simulink model "thermal_control_hardware"  (R2026a)
settings: Solver=FixedStepDiscrete  StopTime=inf  FixedStep=0.1  EnableMultiTasking=on
libraries: slpidlib x1
settings Model: SimulationMode=external  SILPILModeSetting=veronly  ExtModeTrigDuration=2  Creator=Fufal Jigar  LastModifiedBy=Fufal Jigar
settings HardwareCC: ProdBitPerInt=16.0  ProdBitPerPointer=16.0  ProdBitPerSizeT=16.0  ProdBitPerPtrDiffT=16.0  ProdWordSize=8.0  ProdHWDeviceType=Atmel->AVR  UseEmbeddedCoderFeatures=off  UseSimulinkCoderFeatures=off
settings RTWCC: SystemTargetFile=ert.tlc  HardwareBoard=Arduino Mega 2560  TLCOptions=-aInlineSetEventsForThisBaseRateFcn=TLC_FALSE -aSuppressMultiTaskScheduler=TLC_FALSE -aRateBasedStepFcn=1  Toolchain=Arduino AVR  BuildConfiguration=Faster Runs  Description=Embedded Coder
settings ERTTargetCC: ExtModeTransport=3.0  ExtModeAutomaticAllocSize=off  ExtModeStaticAllocSize=2048.0  SupportContinuousTime=on  SupportNonInlinedSFcns=on  SupportVariableSizeSignals=on

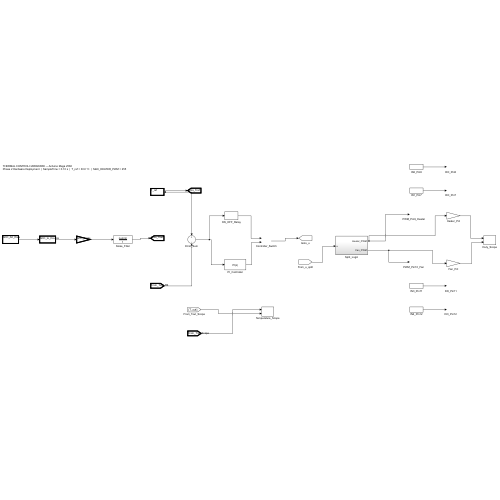
[thumbnail: Simulink's stored preview of the top-level diagram]
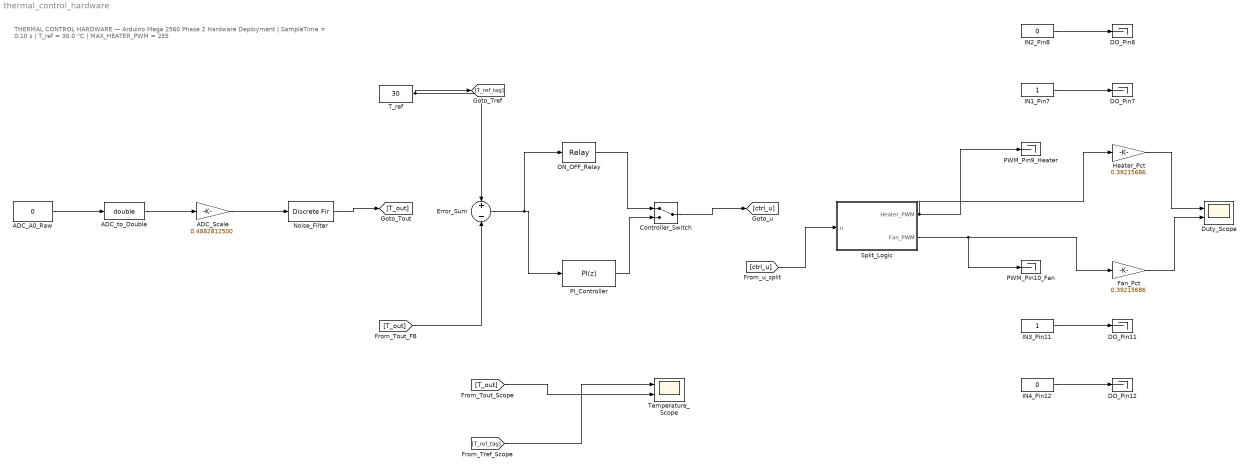
== system thermal_control_hardware ==
  note: THERMAL CONTROL HARDWARE — Arduino Mega 2560
      | Phase 2 Hardware Deployment  |  SampleTime = 0.10 s  |  T_ref = 30.0 °C  |  MAX_HEATER_PWM = 255
  ADC_A0_Raw : Constant  Value=0
  ADC_Scale : Gain  Gain=0.4882812500
  ADC_to_Double : DataTypeConversion  OutDataTypeStr=double  SaturateOnIntegerOverflow=off  RndMeth=Floor
  Controller_Switch : ManualSwitch
  DO_Pin{7..8,11..12} (4 alike) : Terminator
  Duty_Scope : Scope  NumInputPorts=2
  Error_Sum : Sum  Inputs=+-
  Fan_Pct : Gain  Gain=0.39215686
  Heater_Pct : Gain  Gain=0.39215686
  IN1_Pin7 : Constant  OutDataTypeStr=boolean
  IN2_Pin8 : Constant  Value=0  OutDataTypeStr=boolean
  IN3_Pin11 : Constant  OutDataTypeStr=boolean
  IN4_Pin12 : Constant  Value=0  OutDataTypeStr=boolean
  Noise_Filter : DiscreteFir  Coefficients=[0.2 0.2 0.2 0.2 0.2]  SampleTime=0.1
  ON_OFF_Relay : Relay  OnSwitchValue=0.5  OffSwitchValue=-0.5  OnOutputValue=255  OffOutputValue=-255
  PI_Controller : slpidlib/PID Controller  Controller=PI  Form=Parallel  TimeDomain=Discrete-time  UseExternalTs=off  SampleTime=0.1  IntegratorMethod=Forward Euler  FilterMethod=Forward Euler  ControllerParametersSource=internal  P=0.444400  I=0.003700  UseKiTs=off  D=0  UseExternalDerivativeSource=off  N=100  UseFilter=on  TunerSelectOption=Transfer Function Based (PID Tuner App)  InitialConditionSource=internal  InitialConditionForIntegrator=0  InitialConditionForFilter=0  DifferentiatorICPrevScaledInput=0  ExternalReset=none  TrackingMode=off  Kt=1  LimitOutput=off  SatLimitsSource=internal  UpperSaturationLimit=255  LowerSaturationLimit=-255  LinearizeAsGain=off  AntiWindupMode=clamping  Kb=1  LimitIntegrator=off  UpperIntegratorSaturationLimit=inf  LowerIntegratorSaturationLimit=-inf  POutMin=[]  POutMax=[]  IOutMin=[]  IOutMax=[]  DOutMin=[]  DOutMax=[]  NOutMin=[]  NOutMax=[]  SumOutMin=[]  SumOutMax=[]  SaturationOutMin=[]  SaturationOutMax=[]  PParamMin=[]  PParamMax=[]  IParamMin=[]  IParamMax=[]  DParamMin=[]  DParamMax=[]  NParamMin=[]  NParamMax=[]  KbParamMin=[]  KbParamMax=[]  KtParamMin=[]  KtParamMax=[]  KbOutMin=[]  KbOutMax=[]  KtOutMin=[]  KtOutMax=[]  IntegratorOutMin=[]  IntegratorOutMax=[]  FilterOutMin=[]  FilterOutMax=[]  SumI1OutMin=[]  SumI1OutMax=[]  SumI2OutMin=[]  SumI2OutMax=[]  SumI3OutMin=[]  SumI3OutMax=[]  SumI4OutMin=[]  SumI4OutMax=[]  SumDOutMin=[]  SumDOutMax=[]  DifferentiatorOutMin=[]  DifferentiatorOutMax=[]  FilterDiffOutCoefMin=[]  FilterDiffOutCoefMax=[]  ReciprocalOutMin=[]  ReciprocalOutMax=[]  SumDenOutMin=[]  SumDenOutMax=[]  SumNumOutMin=[]  SumNumOutMax=[]  DivideOutMin=[]  DivideOutMax=[]  UdiffTsProdOutMin=[]  UdiffTsProdOutMax=[]  NTsProdOutMin=[]  NTsProdOutMax=[]  UintegralTsProdOutMin=[]  UintegralTsProdOutMax=[]  UngainTsProdOutMin=[]  UngainTsProdOutMax=[]  ClampingZeroOutDataTypeStr=Inherit: Inherit via back propagation  ClampingZeroOutMin=[]  ClampingZeroOutMax=[]  FilterDenConstantOutDataTypeStr=Inherit: Inherit via back propagation  FilterDenConstantOutMin=[]  FilterDenConstantOutMax=[]  PCopyOutDataTypeStr=Inherit: Inherit via back propagation  PCopyOutMin=[]  PCopyOutMax=[]  NCopyOutDataTypeStr=Inherit: Inherit via back propagation  NCopyOutMin=[]  NCopyOutMax=[]  IntegratorContinuousStateAttributes=''  IntegratorStateMustResolveToSignalObject=off  IntegratorRTWStateStorageClass=Auto  FilterContinuousStateAttributes=''  FilterStateMustResolveToSignalObject=off  FilterRTWStateStorageClass=Auto  ParallelPVariant=InternalParameters  IdealPVariant=Disabled  IVariant=InternalParameters  DVariant=Disabled  IntegratorVariant=Discrete  SatVariant=Disabled  AWVariant=Passthrough  PCopyVariant=Disabled  TRVariant=Disabled  FdbkBlocksVariant=Forward  IdealPFdbkVariant=Disabled  SatFdbkVariant=Disabled  DerivativeFilterVariant=Disabled  NVariant=Disabled  NCopyVariant=Disabled_SignalSpec  FilterICVariant=Disabled  IntegratorICVariant=InternalICs  ExternalResetVariant=Disabled  TRSumVariant=Passthrough  SumFdbkVariant=Disabled  SumVariant=Sum_PI  TsampFilterVariant=InternalTs  TsampNgainVariant=Passthrough  TsampIntegralVariant=Disabled_SignalSpec  ExternalSaturationOutDataTypeStr=Inherit: Same as second input  DerivativeSourceVariant=Disabled  PreIntVariant=InternalPreInt
      settings: LibrarySourceBlock=simulink/Discrete/Discrete PID Controller
  PWM_Pin10_Fan : Terminator
  PWM_Pin9_Heater : Terminator
  Split_Logic : Subsystem
  T_ref : Constant  Value=30
  Temperature_Scope : Scope  NumInputPorts=2
  wires:
  ADC_A0_Raw/1 -> ADC_to_Double/1
  ADC_to_Double/1 -> ADC_Scale/1
  ADC_Scale/1 -> Noise_Filter/1
  Noise_Filter/1 -> [T_out]
  T_ref/1 -> Error_Sum/1, [T_ref_tag]
  [T_out] -> Error_Sum/2
  Error_Sum/1 -> ON_OFF_Relay/1, PI_Controller/1
  ON_OFF_Relay/1 -> Controller_Switch/1
  PI_Controller/1 -> Controller_Switch/2
  Controller_Switch/1 -> [ctrl_u]
  [ctrl_u] -> Split_Logic/1(u)
  IN1_Pin7/1 -> DO_Pin7/1
  IN2_Pin8/1 -> DO_Pin8/1
  IN3_Pin11/1 -> DO_Pin11/1
  IN4_Pin12/1 -> DO_Pin12/1
  Split_Logic/1(Heater_PWM) -> PWM_Pin9_Heater/1, Heater_Pct/1
  Split_Logic/2(Fan_PWM) -> PWM_Pin10_Fan/1, Fan_Pct/1
  [T_ref_tag] -> Temperature_Scope/1
  [T_out] -> Temperature_Scope/2
  Heater_Pct/1 -> Duty_Scope/1
  Fan_Pct/1 -> Duty_Scope/2

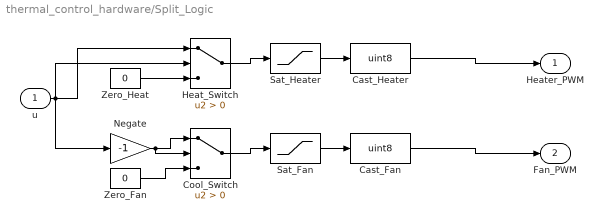
== system thermal_control_hardware/Split_Logic ==
  u : Inport
  Cast_Fan : DataTypeConversion  OutDataTypeStr=uint8  SaturateOnIntegerOverflow=off  RndMeth=Floor
  Cast_Heater : DataTypeConversion  OutDataTypeStr=uint8  SaturateOnIntegerOverflow=off  RndMeth=Floor
  Cool_Switch : Switch  Criteria=u2 > Threshold  SaturateOnIntegerOverflow=off  InputSameDT=off
  Heat_Switch : Switch  Criteria=u2 > Threshold  SaturateOnIntegerOverflow=off  InputSameDT=off
  Negate : Gain  Gain=-1
  Sat_Fan : Saturate  UpperLimit=255  LowerLimit=0
  Sat_Heater : Saturate  UpperLimit=255  LowerLimit=0
  Zero_Fan : Constant  Value=0
  Zero_Heat : Constant  Value=0
  Heater_PWM : Outport
  Fan_PWM : Outport  Port=2
  wires:
  u/1 -> Heat_Switch/1, Heat_Switch/2, Negate/1
  Zero_Heat/1 -> Heat_Switch/3
  Heat_Switch/1 -> Sat_Heater/1
  Sat_Heater/1 -> Cast_Heater/1
  Cast_Heater/1 -> Heater_PWM/1
  Negate/1 -> Cool_Switch/1, Cool_Switch/2
  Zero_Fan/1 -> Cool_Switch/3
  Cool_Switch/1 -> Sat_Fan/1
  Sat_Fan/1 -> Cast_Fan/1
  Cast_Fan/1 -> Fan_PWM/1
